simulink model "eml_hdl_design_patterns"  (R2026a)
settings: Solver=FixedStepDiscrete  StopTime=10
InitFcn:
  | errMsg  = ['\n\nThis model is only for demonstration purposes.\n\nPlease do not Simulate or code generate directly from this model. \n\nBefore generating code from this model please do copy the relevant blocks of interest from this model to a new model, place them in a subsystem, build a valid test bench around them.\n\nPlease refer to the example model ''eml_hdl_incrementer'' or HDLCoder documentation'];
  | error(sprintf(errMsg));
undefined symbols (not defined in the file or in its folder): C, gain_val, init_val, lower_limit, maxWordLength, thresh, upper_limit
libraries: simulink x2
(part 2 of 5)

== matlab function eml_hdl_design_patterns/Counters/counter_up_down_enable ==
  settings: fimath=|
      | fimath(...
      | 'RoundMode', 'floor',...
      | 'OverflowMode', 'wrap',...
      | 'ProductMode', 'FullPrecision', 'ProductWordLength', 32,...
      | 'SumMode', 'FullPrecision', 'SumWordLength', 32,...
      | 'CastBeforeSum', true)
  data: count output fixdt(0,4,0) size=1; up input boolean; down input boolean
function count = fcn(up, down)

% synchronous up down counter
% If "up" is set, it counts up.
% Else, if "down" is set, it counts down
% If neither is set it's disabled.

result_nt = numerictype(0,4,0);

% With "saturate" set this counter will never rollover.  To make it
% rollover, set the 'OverflowMode' to 'wrap'.
result_fm = fimath('OverflowMode', 'saturate', 'RoundMode', 'floor');

persistent count_reg;
if isempty(count_reg)
    count_reg = fi(0, result_nt, result_fm);
end

count = count_reg;

if up   
    inc = count_reg + fi(1, result_nt, result_fm);
    count_reg = fi(inc, result_nt, result_fm);
elseif down
    dec = count_reg - fi(1, result_nt, result_fm);
    count_reg = fi(dec, result_nt, result_fm);
end

== matlab function eml_hdl_design_patterns/Adders/full_adder ==
  settings: fimath=|
      | fimath(...
      | 'RoundMode', 'floor',...
      | 'OverflowMode', 'wrap',...
      | 'ProductMode', 'FullPrecision', 'ProductWordLength', 32,...
      | 'SumMode', 'FullPrecision', 'SumWordLength', 32,...
      | 'CastBeforeSum', true)
  data: a input fixdt(0,1,0); sum output; b input fixdt(0,1,0); cin input fixdt(0,1,0); cout output
function [sum,cout] = fcn(a, b, cin)

% Full Adder

% sum = (a^b)^cin
sum1 = bitxor(a,  b);
sum = bitxor(sum1, cin);

% cout = (a & b) | (b & cin) | (a & cin);
cout = bitor(bitor(bitand(a, b), bitand(b, cin)), bitand(a, cin));

== matlab function eml_hdl_design_patterns/Adders/unsigned_adder ==
  settings: fimath=|
      | fimath(...
      | 'RoundMode', 'floor',...
      | 'OverflowMode', 'wrap',...
      | 'ProductMode', 'FullPrecision', 'ProductWordLength', 32,...
      | 'SumMode', 'FullPrecision', 'SumWordLength', 32,...
      | 'CastBeforeSum', true)
  data: a input fixdt(0,3,0); sum output; b input fixdt(0,3,0)
function sum  = fcn(a, b)

% check default fimath settings on the block
% that define the following unsigned addition semantics
sum = a + b;

== matlab function eml_hdl_design_patterns/Adders/add_with_carry ==
  settings: fimath=|
      | fimath(...
      | 'RoundMode', 'floor',...
      | 'OverflowMode', 'wrap',...
      | 'ProductMode', 'FullPrecision', 'ProductWordLength', 32,...
      | 'SumMode', 'FullPrecision', 'SumWordLength', 32,...
      | 'CastBeforeSum', true)
  data: u1 input fixdt(1,5,0); sum output; u2 input fixdt(1,5,0); carry output; overflow output; c_in input fixdt(0,1,0); flags output
function [sum,carry,overflow,flags] = fcn(u1,u2,c_in)

% add with carry
% generates various CPU flags found in a FLAG register

nt_u1 = numerictype(u1);
fm_u1 = fimath(u1);

wlen  = nt_u1.WordLength;
ufix1_nt = numerictype(0, 1, 0);

% zero extend u1 by a bit
t_u1 = fi(u1, 1, wlen+1, 0);
t_u1 = bitset(t_u1, wlen+1, 0);

% zero extend u2 by a bit
t_u2 = fi(u2, 1, wlen+1, 0);
t_u2 = bitset(t_u2, wlen+1, 0);

% perform the addition
temp_sum = fi(t_u1+t_u2+c_in, 1, wlen+1, 0, fm_u1);

% Carry Flag (get msb)
carry = bitsliceget(temp_sum, wlen+1, wlen+1);

% Extract actual Sum
sum = fi(temp_sum, 1, wlen, 0, fm_u1);

% Negativity flag (N)
msb = getmsb(sum);

% Overflow Flag (V)
u1msb = getmsb(u1);
u2msb = getmsb(u2);
if((u1msb == u2msb) && (msb ~= u1msb))
    overflow = fi(1, ufix1_nt, fm_u1);
else
    overflow = fi(0, ufix1_nt, fm_u1);
end

if (all(sum))    
    zero = fi(1, 0, 1, 0);
else
    zero = fi(0, 0, 1, 0);
end

 
% construct the flag register
% flags = 'C N V Z'
flags = bitconcat(bitconcat(bitconcat(carry, msb), overflow), zero);

== matlab function eml_hdl_design_patterns/Adders/sub_with_borrow ==
  settings: fimath=|
      | fimath(...
      | 'RoundMode', 'floor',...
      | 'OverflowMode', 'wrap',...
      | 'ProductMode', 'FullPrecision', 'ProductWordLength', 32,...
      | 'SumMode', 'FullPrecision', 'SumWordLength', 32,...
      | 'CastBeforeSum', true)
  data: diff output; borrow output; u1 input fixdt(1,5,0); u2 input fixdt(1,5,0); overflow output; c_in input fixdt(0,1,0); flags output
function [diff,borrow,overflow,flags] = fcn(u1,u2,c_in)
% Implement add with carry using subtract with borrow

[diff,borrow,overflow,flags] = add_w_carry(u1,bitcmp(u2),bitcmp(c_in));


function [sum,carry,overflow,flags] = add_w_carry(u1,u2,c_in)

% add with carry
% generates various CPU flags found in a FLAG register

nt_u1 = numerictype(u1);
fm_u1 = fimath(u1);

wlen  = nt_u1.WordLength;
ufix1_nt = numerictype(0, 1, 0);

% zero extend u1 by a bit
t_u1 = fi(u1, 1, wlen+1, 0);
t_u1 = bitset(t_u1, wlen+1, 0);

% zero extend u2 by a bit
t_u2 = fi(u2, 1, wlen+1, 0);
t_u2 = bitset(t_u2, wlen+1, 0);

% perform the addition
temp_sum = fi(t_u1+t_u2+c_in, 1, wlen+1, 0, fm_u1);

% Carry Flag (get msb)
carry = bitsliceget(temp_sum, wlen+1, wlen+1);

% Extract actual Sum
sum = fi(temp_sum, 1, wlen, 0, fm_u1);

% Negativity flag (N)
msb = getmsb(sum);

% Overflow Flag (V)
u1msb = getmsb(u1);
u2msb = getmsb(u2);
if((u1msb == u2msb) && (msb ~= u1msb))
    overflow = fi(1, ufix1_nt, fm_u1);
else
    overflow = fi(0, ufix1_nt, fm_u1);
end

if (all(sum))    
    zero = fi(1, 0, 1, 0);
else
    zero = fi(0, 0, 1, 0);
end

 
% construct the flag register
% flags = 'C N V Z'
flags = bitconcat(bitconcat(bitconcat(carry, msb), overflow), zero);

== matlab function eml_hdl_design_patterns/Shift Registers/shift_reg_1by32 ==
  settings: fimath=|
      | fimath(...
      | 'RoundMode', 'floor',...
      | 'OverflowMode', 'wrap',...
      | 'ProductMode', 'FullPrecision', 'ProductWordLength', 32,...
      | 'SumMode', 'FullPrecision', 'SumWordLength', 32,...
      | 'CastBeforeSum', true)
  data: shift input boolean; sr_out output fixdt(0,1,0); sr_in input fixdt(0,1,0)
function sr_out = fcn(shift, sr_in)
%shift register 1 by 32

persistent sr;
if isempty(sr)
    sr = fi(0, 0, 32, 0, 'fimath', fimath(sr_in));
end

% return sr[31]
sr_out = getmsb(sr);

if (shift)
    % sr_new[32:1] = sr[31:1] & sr_in
    sr = bitconcat(bitsliceget(sr, 31, 1), sr_in);
end

== matlab function eml_hdl_design_patterns/FSMs/moore_fsm ==
  settings: fimath=|
      | fimath(...
      | 'RoundMode', 'nearest',...
      | 'OverflowMode', 'saturate',...
      | 'ProductMode', 'FullPrecision', 'ProductWordLength', 128,...
      | 'SumMode', 'FullPrecision', 'SumWordLength', 128,...
      | 'CastBeforeSum', true)
  data: A input boolean; Z output boolean size=1
function Z = fcn(A)

persistent moore_state_reg;
if isempty(moore_state_reg)
    moore_state_reg = fi(0, 0, 2, 0);   
end

S1 = 0;
S2 = 1;
S3 = 2;
S4 = 3;

switch (moore_state_reg)
    
    case S1
        
        Z = true;
        if (~A)
            moore_state_reg(1) = S1;
        else
            moore_state_reg(1) = S2;
        end
        
    case S2
        
        Z = false;
        if (~A)
            moore_state_reg(1) = S1;
        else
            moore_state_reg(1) = S2;
        end
        
    case S3
        
        Z = false;
        if (~A)
            moore_state_reg(1) = S2;
        else
            moore_state_reg(1) = S3;
        end
        
    case S4
        
        Z = true;
        if (~A)
            moore_state_reg(1) = S1;
        else
            moore_state_reg(1) = S3;
        end
    otherwise
        Z = false;
end

== matlab function eml_hdl_design_patterns/Shift Registers/shift_reg_1by64 ==
  settings: fimath=|
      | fimath(...
      | 'RoundMode', 'floor',...
      | 'OverflowMode', 'wrap',...
      | 'ProductMode', 'FullPrecision', 'ProductWordLength', 32,...
      | 'SumMode', 'FullPrecision', 'SumWordLength', 32,...
      | 'CastBeforeSum', true)
  data: shift input boolean; sr_tap1 output fixdt(0,1,0); sr_in input fixdt(0,1,0); sr_tap2 output
function [sr_tap1,sr_tap2] = fcn(shift, sr_in)

% mimimcing 64bit shift reg, using 32bit word due to
% our fixpt 32bit limitation.

persistent sr_lsw;
persistent sr_msw;

if isempty(sr_lsw)
    sr_lsw = fi(0, 0, 32, 0, 'fimath', fimath(sr_in));
    sr_msw = fi(0, 0, 32, 0, 'fimath', fimath(sr_in));    
end

% return sr_lsw[31]
sr_tap1 = getmsb(sr_lsw);
% return sr_msw[31]
sr_tap2 = getmsb(sr_msw);

if (shift)
    % sr_msw[31:1] = sr_msw[30:0] & sl_lsw[31]
    sr_msw = bitconcat(bitsliceget(sr_msw, 31, 1), getmsb(sr_lsw));
    % sr_lsw[31:1] = sr_lsw[30:0] & sr_in
    sr_lsw = bitconcat(bitsliceget(sr_lsw, 31, 1), sr_in);    
end

== matlab function eml_hdl_design_patterns/Signal Analysis/conv_output_side ==
  settings: fimath=|
      | fimath(...
      | 'RoundMode', 'floor',...
      | 'OverflowMode', 'wrap',...
      | 'ProductMode', 'FullPrecision', 'ProductWordLength', 32,...
      | 'SumMode', 'FullPrecision', 'SumWordLength', 32,...
      | 'CastBeforeSum', true)
  data: u input fixdt(0,6,2) size=80; y output; h input fixdt(0,6,2) size=30
function y = fcn(u, h)

% Convolution: on the output side

% this algorithm specifies how each sample in the output 
% signal can be calculated independently of all other samples 
% in the output signal.

% y has to be fully specified before indexing into it.
%  length(y) == 112, typeof(y) == ufix12_En6

nt = numerictype(0, 12, 6);
fm = fimath(u);

y = fi(zeros(1, 110), nt, fm);

for ii=1:110
    for jj=1:30
        kk = ii - jj;
        if kk >= 1 && kk <= 80
            y(kk) = fi(y(kk) + fi(h(jj) * u(kk), nt, fm), nt, fm);
        end
    end
end

== matlab function eml_hdl_design_patterns/Combinatorics/count_ones_blk ==
  settings: fimath=|
      | fimath(...
      | 'RoundMode', 'floor',...
      | 'OverflowMode', 'wrap',...
      | 'ProductMode', 'FullPrecision', 'ProductWordLength', 32,...
      | 'SumMode', 'FullPrecision', 'SumWordLength', 32,...
      | 'CastBeforeSum', true)
  data: datain input fixdt(0,17,0); result output fixdt(0,18,0) size=1
function result  = fcn(datain)

t = count_bits_in_range(datain);

r_nt = numerictype(0, 18, 0); 
r_fm = fimath('OverflowMode', 'saturate', 'RoundMode', 'floor');

result = fi(t, r_nt, r_fm);

%%%%%%%%%%%%%%%%%%%%%%%%%%%%%%%%%%%%%
% subfunction, counts bits in range
%%%%%%%%%%%%%%%%%%%%%%%%%%%%%%%%%%%%%
function cntOnes = count_bits_in_range(datain)

lbound = 1;
rbound = 17; % wlen of datain

cntOnes = uint8(0);

for ii=lbound:1:rbound
    bit = bitget(datain, ii);
    if logical(bit)
        cntOnes = cntOnes + 1;
    end
end

== matlab function eml_hdl_design_patterns/Misc/saturate_input ==
  data: u input; y output
function y = fcn(u) 
% Implementation of Saturation block with MATLAB code.

% Note Input can be integer or fixedpoint type 
% (see this block setting: treat input as int or fi)


upper_limit = fi(500, numerictype(u), fimath(u));
lower_limit = fi(-500, numerictype(u), fimath(u));

if (u > upper_limit)
    y = upper_limit;
elseif (u < lower_limit)
    y = lower_limit;
else
    y = u;
end

== matlab function eml_hdl_design_patterns/Word Twiddlers/nibble_swap_with_bitops ==
  settings: fimath=|
      | fimath(...
      | 'RoundMode', 'floor',...
      | 'OverflowMode', 'wrap',...
      | 'ProductMode', 'FullPrecision', 'ProductWordLength', 32,...
      | 'SumMode', 'FullPrecision', 'SumWordLength', 32,...
      | 'CastBeforeSum', true)
  data: u input fixdt(0,8,0); y output
function y = fcn(u)
% NIBBLE SWAP (using traditional bitops)

% assumes u is of type ufix8
% lmask = 0x0F
lmask = fi(15, 0, 8, 0, 'fimath', fimath(u));
% lmask = 0xF0
umask = bitsll(lmask, 4);
% mask upper nibble
l_nibble = bitand(u, lmask);
% mask lower nibble
u_nibble = bitand(u, umask);
% shift lower nibble left
ls = bitsll(l_nibble, 4);
% shift upper nibble right
ur = bitsrl(u_nibble, 4);
% final output
y = bitor(ls, ur);

== matlab function eml_hdl_design_patterns/Word Twiddlers/nibble_swap_with_slice_concat ==
  settings: fimath=|
      | fimath(...
      | 'RoundMode', 'floor',...
      | 'OverflowMode', 'wrap',...
      | 'ProductMode', 'FullPrecision', 'ProductWordLength', 32,...
      | 'SumMode', 'FullPrecision', 'SumWordLength', 32,...
      | 'CastBeforeSum', true)
  data: u input fixdt(0,8,0); y output
function y = fcn(u)
% NIBBLE SWAP
y = bitconcat(bitsliceget(u, 4, 1), bitsliceget(u, 8, 5));

== matlab function eml_hdl_design_patterns/Bit Twiddlers/hdl_bit_ops ==
  settings: fimath=|
      | fimath(...
      | 'RoundMode', 'floor',...
      | 'OverflowMode', 'saturate',...
      | 'ProductMode', 'FullPrecision', 'ProductWordLength', 32,...
      | 'SumMode', 'FullPrecision', 'SumWordLength', 32,...
      | 'CastBeforeSum', true)
  data: a input fixdt(0,31,0); b input fixdt(0,31,0); bget output; bslice output; bmsb output; blsb output; bset output; bcmp output; band output; bor output; bxor output; bnand output; bnor output; bnxor output; blshift output; brshift output; band_red output; bor_red output; bxor_red output; bnand_red output; bnor_red output; bnxor_red output
function [...
    bget, bslice, bmsb, blsb,...
    bset, bcmp,...
    band, bor, bxor, ...
    bnand, bnor, bnxor, ...
    blshift, brshift,  ...
    band_red, bor_red, bxor_red, ...
    bnand_red, bnor_red, bnxor_red] = fcn(a,b)


% BITGET
% get bit at position of fixed point input var 'a'
% this uses slice operator in HDL
bget = bitget(a,2);
bslice = bitsliceget(a, 25, 20);
bmsb = getmsb(a);
blsb = getlsb(a);

% BITCLEAR
% clear bit at position 3 and compute new value into 't2'
t2 = bitset(a,3,0);

% BITSET
% now set bit4 in t2
% you need to assign the result back to 't2' to update the variable
bset = bitset(t2,4,1);

% BITCMP
bcmp = bitcmp(a);

% BITAND
band = bitand(a,b);
% BITOR
bor = bitor(a,b);
% BITXOR
bxor = bitxor(a,b);

% BITNAND
bnand = bitcmp(bitand(a,b));
% BITNOR
bnor = bitcmp(bitor(a,b));
% NOT BITXOR
bnxor = bitcmp(bitxor(a,b));

% BITSHIFT
% multitply by 2
blshift = bitsll(a,1); 
% divide by 2
brshift = bitsrl(a,1); 

% AND, XOR, OR REDUCTION 
band_red = bitandreduce(a);
bxor_red = bitxorreduce(a);
bor_red = bitorreduce(a);

% NAND, NOR, NOT XOR, REDUCTION 
bnand_red = bitcmp(band_red);
bnxor_red = bitcmp(bxor_red);
bnor_red = bitcmp(bor_red);

== matlab function eml_hdl_design_patterns/Shift Registers/shift_reg_universal ==
  settings: fimath=|
      | fimath(...
      | 'RoundMode', 'nearest',...
      | 'OverflowMode', 'saturate',...
      | 'ProductMode', 'FullPrecision', 'ProductWordLength', 128,...
      | 'SumMode', 'FullPrecision', 'SumWordLength', 128,...
      | 'CastBeforeSum', true)
  data: Clear input boolean; Q output fixdt(0,3,0) size=1; LeftIn input boolean; RightIn input boolean; S1 input boolean; S2 input boolean; InData input fixdt(0,3,0)
function Q = fcn(Clear, LeftIn, RightIn, S1, S2, InData)

% 3bit universal shift register. it can
%  a) hold value
%  b) shift left
%  c) shift right
%  d) load value

% this can be used as
%  serial-in, serial-out shift reg
%  parallel-in, serial-out shift reg
%  serial-in, parallel-out shift reg
%  parallel-in, parallel-out shift reg

% state table

% --------------------------------------------------------
% function        inputs          next state
%                 S1, S2          Q2 Q1 Q0
% --------------------------------------------------------
% hold            0   0           Q2      Q1      Q0
% shift left      0   1           Q1      Q0      RightIn
% shift right     1   0           LeftIn  Q2      Q1
% load            1   1           in2     in1     in0
% --------------------------------------------------------

persistent Q_reg;
if isempty(Q_reg)
    Q_reg = fi(0, 0, 3, 0);
end

Q = Q_reg;
if Clear
    Q = fi(0, 0, 3, 0);
else
    switch uint8(S1)

        case 0
            switch uint8(S2)
                case 0
                    % state: 00
                    % do nothing
                case 1
                    % state: 01
                    % shift left, and feed datain from right
                    Q_reg = bitsll(Q_reg, 1);
                    Q_reg = bitset(Q_reg, 1, RightIn);
            end

        case 1
            switch uint8(S2)
                case 0
                    % state: 10
                    % shift right, and feed datain from left
                    Q_reg = bitsrl(Q_reg, 1);
                    Q_reg = bitset(Q_reg, 3, LeftIn);
                case 1
                    % state: 11
                    % load value
                    Q_reg = InData;
            end
    end
end

== matlab function eml_hdl_design_patterns/Decoders/monlithic_viterbi ==
  settings: fimath=|
      | fimath(...
      | 'RoundMode', 'floor',...
      | 'OverflowMode', 'wrap',...
      | 'ProductMode', 'FullPrecision', 'ProductWordLength', 32,...
      | 'SumMode', 'FullPrecision', 'SumWordLength', 32,...
      | 'CastBeforeSum', true)
  data: u input fixdt(1,6,3) size=2; y output boolean
function y = fcn(u)
%--------------------------------------------------------------------------
% Viterbi Decoder Demo
% 
% This model implements viterbi decoder with a MATLAB Function Block.
% The Viterbi Decoder block decodes fixed-point input symbols to produce 
% binary output symbols.
%--------------------------------------------------------------------------

% stored paths metrics register
persistent sm_reg;  
if isempty(sm_reg)
    sm_reg = getfi_sat(zeros(1,64),1, 12, 6);
end

% traceback storage register
persistent tb_reg;  
if isempty(tb_reg)
    tb_reg = getfi(zeros(1,64), 0, 27, 0);
end

% traceback output register
persistent tbout_reg
if isempty(tbout_reg)
    tbout_reg = getfi(0,0,1,0);
end

% input symbol
u1 = u(1);
u2 = u(2);

%--------------------------------------------------------------------------
% BMC (Branch Metric) Unit
% This block calculates the Branch Metric (Hamming distance) of input symbols.
% The input are the quantized fixed-point symbols in the form of sfix6_En3.
%--------------------------------------------------------------------------
bm = getfi_sat(zeros(1,4), 1, 12, 6);

%----------------------------
% Hamming distace for (1,1)
%----------------------------
bm(1) = (u1-1)*(u1-1) + (u2-1)*(u2-1);

%----------------------------
% Hamming distace for (1,-1)
%----------------------------
bm(2) = (u1-1)*(u1-1) + (u2-(-1))*(u2-(-1));

%----------------------------
% Hamming distace for (-1,1)
%----------------------------
bm(3) = (u1-(-1))*(u1-(-1)) + (u2-1)*(u2-1);

%----------------------------
% Hamming distace for (-1,-1)
%----------------------------
bm(4) = (u1-(-1))*(u1-(-1)) + (u2-(-1))*(u2-(-1));

%--------------------------------------------------------------------------
% PMU (Path Metric Unit)
% This block calculates and compares the path metrics to get the optimal path.
% The core elements of this block are 
%  a) ACS (Add-Compare-Select) block, and 
%  b) Renormalize block
%--------------------------------------------------------------------------

% ACS Unit Group Block
[nsm, dec] = acsunitbutterfly(bm, sm_reg);

% Renormalize Block
% Finds the state with minimum path metric and outputs its index
% Then renormalizes all the path metrics by subsracting the minimum metric
[minimum, idx] = tree_min(nsm);
index = getfi((idx-1), 0, 8, 0);
sm_reg = getfi_sat((nsm - minimum), 1, 12, 6);
    
%--------------------------------------------------------------------------
% TBU (Trace Back Unit)
% Trace back unit restore the optimal path information stored in the 
% path metric register. The trace back depth of this decoder is 32 steps,
% which means every decoded symbol is based on the minimum path metric in the
% following 32 steps. 
%
% The trace back unit is implemented by a 27 stage shift register.
% Only 27 stage is necessary (instead of 32) because we can retrieve the 
% input symbol of the 32th stage from the shift register index of the 27th stage.
%
% Normal implementation uses 27 64-bit registers for trance back unit. 
% We use 64 27-bit registers instead because of the fixed-point bitwidth limit.
%--------------------------------------------------------------------------

% stores path metric decision inforamtion from PMU unit
tb_reg = bitshift(tb_reg, 1);
tb_reg = bitset(tb_reg, ones(1,64), uint8(dec));

% trace back unit
for i=1:27
  index = tbunit(index, tb_reg, i);
end

% the LSB of the 27th trace back step is the decoder output
tbmask = getfi(1, 0, 8, 0);
tband = bitand(index, tbmask);

% register the final result
prev_result = tbout_reg;
tbout_reg = getfi(tband, 0, 1, 0);

% update output as boolean datatype
y =  (prev_result == getfi(1, 0, 1, 0));

end

%--------------------------------------------------------------------------
% TB Unit (Trace Back Unit)
% Given the index of the minimum metric node in the current stages,
% also given the stored decision information in the current stages,
% we can restore the index of the minimum metric node in the previous stage.
%--------------------------------------------------------------------------
function new_idx = tbunit (current_idx, tb_reg, stage)

idx = int8(current_idx) + int8(1);
tbread = bitget(tb_reg(idx), stage);

tbshift = bitshift(current_idx, 1);
tband = bitand(tbshift, getfi(62, 0, 8, 0));
new_idx = bitor(tband, getfi(tbread, 0, 8, 0));

end

%--------------------------------------------------------------------------
% ACS Unit Group(Add-Compare-Select)
% For each state in the trellis diagram, for each node in this state:
% 1. Add the branch metric to the paths merged to this node. 
% 2. Compare all the paths merged to this road
% 3. Select the path with the minimum path metric
%
% The following code is generated by a script 'generateviterbi.m'
% that generates trellis diagram for convolution code (7,171,133)
%--------------------------------------------------------------------------
function [nsm, dec] = acsunitbutterfly(bm, sm)

nsm = getfi(zeros(1,64),1, 12, 6);
dec = getfi(zeros(1,64),0, 1,  0);

%----------------------------------------------------
% 000000   -> 00 -> 000000   000001   -> 11 -> 000000   
%----------------------------------------------------
[nsm(1), dec(1)] = acsunit(bm(1),bm(4),sm(1),sm(2));
%----------------------------------------------------
% 000000   -> 11 -> 100000   000001   -> 00 -> 100000   
%----------------------------------------------------
[nsm(33), dec(33)] = acsunit(bm(4),bm(1),sm(1),sm(2));
%----------------------------------------------------
% 000010   -> 01 -> 000001   000011   -> 10 -> 000001   
%----------------------------------------------------
[nsm(2), dec(2)] = acsunit(bm(2),bm(3),sm(3),sm(4));
%----------------------------------------------------
% 000010   -> 10 -> 100001   000011   -> 01 -> 100001   
%----------------------------------------------------
[nsm(34), dec(34)] = acsunit(bm(3),bm(2),sm(3),sm(4));
%----------------------------------------------------
% 000100   -> 00 -> 000010   000101   -> 11 -> 000010   
%----------------------------------------------------
[nsm(3), dec(3)] = acsunit(bm(1),bm(4),sm(5),sm(6));
%----------------------------------------------------
% 000100   -> 11 -> 100010   000101   -> 00 -> 100010   
%----------------------------------------------------
[nsm(35), dec(35)] = acsunit(bm(4),bm(1),sm(5),sm(6));
%----------------------------------------------------
% 000110   -> 01 -> 000011   000111   -> 10 -> 000011   
%----------------------------------------------------
[nsm(4), dec(4)] = acsunit(bm(2),bm(3),sm(7),sm(8));
%----------------------------------------------------
% 000110   -> 10 -> 100011   000111   -> 01 -> 100011   
%----------------------------------------------------
[nsm(36), dec(36)] = acsunit(bm(3),bm(2),sm(7),sm(8));
%----------------------------------------------------
% 001000   -> 11 -> 000100   001001   -> 00 -> 000100   
%----------------------------------------------------
[nsm(5), dec(5)] = acsunit(bm(4),bm(1),sm(9),sm(10));
%----------------------------------------------------
% 001000   -> 00 -> 100100   001001   -> 11 -> 100100   
%----------------------------------------------------
[nsm(37), dec(37)] = acsunit(bm(1),bm(4),sm(9),sm(10));
%----------------------------------------------------
% 001010   -> 10 -> 000101   001011   -> 01 -> 000101   
%----------------------------------------------------
[nsm(6), dec(6)] = acsunit(bm(3),bm(2),sm(11),sm(12));
%----------------------------------------------------
% 001010   -> 01 -> 100101   001011   -> 10 -> 100101   
%----------------------------------------------------
[nsm(38), dec(38)] = acsunit(bm(2),bm(3),sm(11),sm(12));
%----------------------------------------------------
% 001100   -> 11 -> 000110   001101   -> 00 -> 000110   
%----------------------------------------------------
[nsm(7), dec(7)] = acsunit(bm(4),bm(1),sm(13),sm(14));
%----------------------------------------------------
% 001100   -> 00 -> 100110   001101   -> 11 -> 100110   
%----------------------------------------------------
[nsm(39), dec(39)] = acsunit(bm(1),bm(4),sm(13),sm(14));
%----------------------------------------------------
% 001110   -> 10 -> 000111   001111   -> 01 -> 000111   
%----------------------------------------------------
[nsm(8), dec(8)] = acsunit(bm(3),bm(2),sm(15),sm(16));
%----------------------------------------------------
% 001110   -> 01 -> 100111   001111   -> 10 -> 100111   
%----------------------------------------------------
[nsm(40), dec(40)] = acsunit(bm(2),bm(3),sm(15),sm(16));
%----------------------------------------------------
% 010000   -> 11 -> 001000   010001   -> 00 -> 001000   
%----------------------------------------------------
[nsm(9), dec(9)] = acsunit(bm(4),bm(1),sm(17),sm(18));
%----------------------------------------------------
% 010000   -> 00 -> 101000   010001   -> 11 -> 101000   
%----------------------------------------------------
[nsm(41), dec(41)] = acsunit(bm(1),bm(4),sm(17),sm(18));
%----------------------------------------------------
% 010010   -> 10 -> 001001   010011   -> 01 -> 001001   
%----------------------------------------------------
[nsm(10), dec(10)] = acsunit(bm(3),bm(2),sm(19),sm(20));
%----------------------------------------------------
% 010010   -> 01 -> 101001   010011   -> 10 -> 101001   
%----------------------------------------------------
[nsm(42), dec(42)] = acsunit(bm(2),bm(3),sm(19),sm(20));
%----------------------------------------------------
% 010100   -> 11 -> 001010   010101   -> 00 -> 001010   
%----------------------------------------------------
[nsm(11), dec(11)] = acsunit(bm(4),bm(1),sm(21),sm(22));
%----------------------------------------------------
% 010100   -> 00 -> 101010   010101   -> 11 -> 101010   
%----------------------------------------------------
[nsm(43), dec(43)] = acsunit(bm(1),bm(4),sm(21),sm(22));
%----------------------------------------------------
% 010110   -> 10 -> 001011   010111   -> 01 -> 001011   
%----------------------------------------------------
[nsm(12), dec(12)] = acsunit(bm(3),bm(2),sm(23),sm(24));
%----------------------------------------------------
% 010110   -> 01 -> 101011   010111   -> 10 -> 101011   
%----------------------------------------------------
[nsm(44), dec(44)] = acsunit(bm(2),bm(3),sm(23),sm(24));
%----------------------------------------------------
% 011000   -> 00 -> 001100   011001   -> 11 -> 001100   
%----------------------------------------------------
[nsm(13), dec(13)] = acsunit(bm(1),bm(4),sm(25),sm(26));
%----------------------------------------------------
% 011000   -> 11 -> 101100   011001   -> 00 -> 101100   
%----------------------------------------------------
[nsm(45), dec(45)] = acsunit(bm(4),bm(1),sm(25),sm(26));
%----------------------------------------------------
% 011010   -> 01 -> 001101   011011   -> 10 -> 001101   
%----------------------------------------------------
[nsm(14), dec(14)] = acsunit(bm(2),bm(3),sm(27),sm(28));
%----------------------------------------------------
% 011010   -> 10 -> 101101   011011   -> 01 -> 101101   
%----------------------------------------------------
[nsm(46), dec(46)] = acsunit(bm(3),bm(2),sm(27),sm(28));
%----------------------------------------------------
% 011100   -> 00 -> 001110   011101   -> 11 -> 001110   
%----------------------------------------------------
[nsm(15), dec(15)] = acsunit(bm(1),bm(4),sm(29),sm(30));
%----------------------------------------------------
% 011100   -> 11 -> 101110   011101   -> 00 -> 101110   
%----------------------------------------------------
[nsm(47), dec(47)] = acsunit(bm(4),bm(1),sm(29),sm(30));
%----------------------------------------------------
% 011110   -> 01 -> 001111   011111   -> 10 -> 001111   
%----------------------------------------------------
[nsm(16), dec(16)] = acsunit(bm(2),bm(3),sm(31),sm(32));
%----------------------------------------------------
% 011110   -> 10 -> 101111   011111   -> 01 -> 101111   
%----------------------------------------------------
[nsm(48), dec(48)] = acsunit(bm(3),bm(2),sm(31),sm(32));
%----------------------------------------------------
% 100000   -> 10 -> 010000   100001   -> 01 -> 010000   
%----------------------------------------------------
[nsm(17), dec(17)] = acsunit(bm(3),bm(2),sm(33),sm(34));
%----------------------------------------------------
% 100000   -> 01 -> 110000   100001   -> 10 -> 110000   
%----------------------------------------------------
[nsm(49), dec(49)] = acsunit(bm(2),bm(3),sm(33),sm(34));
%----------------------------------------------------
% 100010   -> 11 -> 010001   100011   -> 00 -> 010001   
%----------------------------------------------------
[nsm(18), dec(18)] = acsunit(bm(4),bm(1),sm(35),sm(36));
%----------------------------------------------------
% 100010   -> 00 -> 110001   100011   -> 11 -> 110001   
%----------------------------------------------------
[nsm(50), dec(50)] = acsunit(bm(1),bm(4),sm(35),sm(36));
%----------------------------------------------------
% 100100   -> 10 -> 010010   100101   -> 01 -> 010010   
%----------------------------------------------------
[nsm(19), dec(19)] = acsunit(bm(3),bm(2),sm(37),sm(38));
%----------------------------------------------------
% 100100   -> 01 -> 110010   100101   -> 10 -> 110010   
%----------------------------------------------------
[nsm(51), dec(51)] = acsunit(bm(2),bm(3),sm(37),sm(38));
%----------------------------------------------------
% 100110   -> 11 -> 010011   100111   -> 00 -> 010011   
%----------------------------------------------------
[nsm(20), dec(20)] = acsunit(bm(4),bm(1),sm(39),sm(40));
%----------------------------------------------------
% 100110   -> 00 -> 110011   100111   -> 11 -> 110011   
%----------------------------------------------------
[nsm(52), dec(52)] = acsunit(bm(1),bm(4),sm(39),sm(40));
%----------------------------------------------------
% 101000   -> 01 -> 010100   101001   -> 10 -> 010100   
%----------------------------------------------------
[nsm(21), dec(21)] = acsunit(bm(2),bm(3),sm(41),sm(42));
%----------------------------------------------------
% 101000   -> 10 -> 110100   101001   -> 01 -> 110100   
%----------------------------------------------------
[nsm(53), dec(53)] = acsunit(bm(3),bm(2),sm(41),sm(42));
%----------------------------------------------------
% 101010   -> 00 -> 010101   101011   -> 11 -> 010101   
%----------------------------------------------------
[nsm(22), dec(22)] = acsunit(bm(1),bm(4),sm(43),sm(44));
%----------------------------------------------------
% 101010   -> 11 -> 110101   101011   -> 00 -> 110101   
%----------------------------------------------------
[nsm(54), dec(54)] = acsunit(bm(4),bm(1),sm(43),sm(44));
%----------------------------------------------------
% 101100   -> 01 -> 010110   101101   -> 10 -> 010110   
%----------------------------------------------------
[nsm(23), dec(23)] = acsunit(bm(2),bm(3),sm(45),sm(46));
%----------------------------------------------------
% 101100   -> 10 -> 110110   101101   -> 01 -> 110110   
%----------------------------------------------------
[nsm(55), dec(55)] = acsunit(bm(3),bm(2),sm(45),sm(46));
%----------------------------------------------------
% 101110   -> 00 -> 010111   101111   -> 11 -> 010111   
%----------------------------------------------------
[nsm(24), dec(24)] = acsunit(bm(1),bm(4),sm(47),sm(48));
%----------------------------------------------------
% 101110   -> 11 -> 110111   101111   -> 00 -> 110111   
%----------------------------------------------------
[nsm(56), dec(56)] = acsunit(bm(4),bm(1),sm(47),sm(48));
%----------------------------------------------------
% 110000   -> 01 -> 011000   110001   -> 10 -> 011000   
%----------------------------------------------------
[nsm(25), dec(25)] = acsunit(bm(2),bm(3),sm(49),sm(50));
%----------------------------------------------------
% 110000   -> 10 -> 111000   110001   -> 01 -> 111000   
%----------------------------------------------------
[nsm(57), dec(57)] = acsunit(bm(3),bm(2),sm(49),sm(50));
%----------------------------------------------------
% 110010   -> 00 -> 011001   110011   -> 11 -> 011001   
%----------------------------------------------------
[nsm(26), dec(26)] = acsunit(bm(1),bm(4),sm(51),sm(52));
%----------------------------------------------------
% 110010   -> 11 -> 111001   110011   -> 00 -> 111001   
%----------------------------------------------------
[nsm(58), dec(58)] = acsunit(bm(4),bm(1),sm(51),sm(52));
%----------------------------------------------------
% 110100   -> 01 -> 011010   110101   -> 10 -> 011010   
%----------------------------------------------------
[nsm(27), dec(27)] = acsunit(bm(2),bm(3),sm(53),sm(54));
%----------------------------------------------------
% 110100   -> 10 -> 111010   110101   -> 01 -> 111010   
%----------------------------------------------------
[nsm(59), dec(59)] = acsunit(bm(3),bm(2),sm(53),sm(54));
%----------------------------------------------------
% 110110   -> 00 -> 011011   110111   -> 11 -> 011011   
%----------------------------------------------------
[nsm(28), dec(28)] = acsunit(bm(1),bm(4),sm(55),sm(56));
%----------------------------------------------------
% 110110   -> 11 -> 111011   110111   -> 00 -> 111011   
%----------------------------------------------------
[nsm(60), dec(60)] = acsunit(bm(4),bm(1),sm(55),sm(56));
%----------------------------------------------------
% 111000   -> 10 -> 011100   111001   -> 01 -> 011100   
%----------------------------------------------------
[nsm(29), dec(29)] = acsunit(bm(3),bm(2),sm(57),sm(58));
%----------------------------------------------------
% 111000   -> 01 -> 111100   111001   -> 10 -> 111100   
%----------------------------------------------------
[nsm(61), dec(61)] = acsunit(bm(2),bm(3),sm(57),sm(58));
%----------------------------------------------------
% 111010   -> 11 -> 011101   111011   -> 00 -> 011101   
%----------------------------------------------------
[nsm(30), dec(30)] = acsunit(bm(4),bm(1),sm(59),sm(60));
%----------------------------------------------------
% 111010   -> 00 -> 111101   111011   -> 11 -> 111101   
%----------------------------------------------------
[nsm(62), dec(62)] = acsunit(bm(1),bm(4),sm(59),sm(60));
%----------------------------------------------------
% 111100   -> 10 -> 011110   111101   -> 01 -> 011110   
%----------------------------------------------------
[nsm(31), dec(31)] = acsunit(bm(3),bm(2),sm(61),sm(62));
%----------------------------------------------------
% 111100   -> 01 -> 111110   111101   -> 10 -> 111110   
%----------------------------------------------------
[nsm(63), dec(63)] = acsunit(bm(2),bm(3),sm(61),sm(62));
%----------------------------------------------------
% 111110   -> 11 -> 011111   111111   -> 00 -> 011111   
%----------------------------------------------------
[nsm(32), dec(32)] = acsunit(bm(4),bm(1),sm(63),sm(64));
%----------------------------------------------------
% 111110   -> 00 -> 111111   111111   -> 11 -> 111111   
%----------------------------------------------------
[nsm(64), dec(64)] = acsunit(bm(1),bm(4),sm(63),sm(64));

end    
    
% ACS unit
function [select_metric, decision] = acsunit(branch_metric0, branch_metric1, stored_metric0, stored_metric1)

    % update branch0 metric
    a = getfi_sat(branch_metric0 + stored_metric0, 1, 12, 6);

    % update branch1 metric
    b = getfi_sat(branch_metric1 + stored_metric1, 1, 12, 6);
    
    % choose the metric
    if (a <= b)
        select_metric = a;
        decision = getfi(0, 0, 1, 0);
    else
        select_metric = b;
        decision = getfi(1, 0, 1, 0);
    end
end
            
%--------------------------------------------------------------------------
% Tree implementation min function for vector input of length 64
%--------------------------------------------------------------------------
function [minval, idx] = tree_min(invec)

% initialize outputs
minval = getfi(0, 1, 12, 6);
idx = 0;

% first level of comparison
inidx = 1:64;
[lvlonemin, lvloneidx] = vector_min(invec, inidx);

% second level of comparison
[lvltwomin, lvltwoidx] = vector_min(lvlonemin, lvloneidx);

% third level of comparison
[lvlthreemin, lvlthreeidx] = vector_min(lvltwomin, lvltwoidx);

% fourth level of comparison
[lvlfourmin, lvlfouridx] = vector_min(lvlthreemin, lvlthreeidx);

% fifth level of comparison
[lvlfivemin, lvlfiveidx] = vector_min(lvlfourmin, lvlfouridx);

% final comparison
[minval, idx] = vector_min(lvlfivemin, lvlfiveidx);

end

% Minimum subfuction for tree implementation
function [minvec, idxvec] = vector_min(invec, inidx)
    
lengthminvec = uint8(length(invec)/2);
minvec = getfi(zeros(lengthminvec, 1), 1, 12, 6);
idxvec = zeros(lengthminvec, 1);

for i=1:lengthminvec
    % get two consecutive values
    idx2 = int8(i)+int8(i); %i*2
    idx1 = int8(idx2) - int8(1); %i*2-1
    % get elements
    val1 = invec(idx1);
    val2 = invec(idx2);
    % compare them and select minimum
    if le(val1, val2)
        minvec(i) = val1;
        idxvec(i) = inidx(idx1);
    else
        minvec(i) = val2;
        idxvec(i) = inidx(idx2);
    end
end

end


function myfi = getfi(input, issigned, wlen, flen)

fm = fimath(...
    'RoundMode', 'floor',...
    'OverflowMode', 'wrap',...
    'ProductMode', 'FullPrecision', 'ProductWordLength', 32,...
    'SumMode', 'FullPrecision', 'SumWordLength', 32,...
    'CastBeforeSum', true);

myfi = fi(input, issigned, wlen, flen, 'fimath', fm);

end


function myfi = getfi_sat(input, issigned, wlen, flen)

fm_sat = fimath(...
    'RoundMode', 'floor',...
    'OverflowMode', 'saturate',...
    'ProductMode', 'FullPrecision', 'ProductWordLength', 32,...
    'SumMode', 'FullPrecision', 'SumWordLength', 32,...
    'CastBeforeSum', true);

myfi = fi(input, issigned, wlen, flen, 'fimath', fm_sat);

end

== matlab function eml_hdl_design_patterns/Mux Demux/demux_using_for_blk ==
  settings: fimath=|
      | fimath(...
      | 'RoundMode', 'floor',...
      | 'OverflowMode', 'wrap',...
      | 'ProductMode', 'FullPrecision', 'ProductWordLength', 32,...
      | 'SumMode', 'FullPrecision', 'SumWordLength', 32,...
      | 'CastBeforeSum', true)
  data: address input uint8; line output fixdt(0,1,0) size=4
function line  = fcn(address)

line = fi(zeros(4, 1), 0, 1, 0);

for J=4:-1:1
    if (address == J)
        line(J) = 1;
    else
        line(J) = 0;
    end
end

== matlab function eml_hdl_design_patterns/Decoders/decoder_n_bit ==
  settings: fimath=|
      | fimath(...
      | 'RoundMode', 'floor',...
      | 'OverflowMode', 'wrap',...
      | 'ProductMode', 'FullPrecision', 'ProductWordLength', 32,...
      | 'SumMode', 'FullPrecision', 'SumWordLength', 32,...
      | 'CastBeforeSum', true)
  data: select_addr input boolean; decode_out output fixdt(0,1,0) size=4
function decode_out  = fcn(select_addr)

% N bit binary decoder

decode_out = fi(zeros(4,1), 0, 1, 0);

for jj = 4 : -1 : 1
    if jj == select_addr
        decode_out(jj) = fi(0, 0, 1, 0);
    else
        decode_out(jj) = fi(1, 0, 1, 0);
    end
end

== matlab function eml_hdl_design_patterns/Decoders/decoder_2_by_4 ==
  settings: fimath=|
      | fimath(...
      | 'RoundMode', 'floor',...
      | 'OverflowMode', 'wrap',...
      | 'ProductMode', 'FullPrecision', 'ProductWordLength', 32,...
      | 'SumMode', 'FullPrecision', 'SumWordLength', 32,...
      | 'CastBeforeSum', true)
  data: a input boolean; decode_out output fixdt(0,4,0) size=1; b input boolean; enable input boolean
function decode_out  = fcn(a, b, enable)

% 2 by 4 decoder circuit.

result_nt = numerictype(0,4,0);
result_fm = fimath('OverflowMode', 'wrap', 'RoundMode', 'floor');
decode_out = fi(0, result_nt, result_fm);

a_bar = ~a;
b_bar = ~b;

% compute bit0
decode_out = bitset(decode_out, 1, ~(enable & a_bar & b_bar));
% compute bit1
decode_out = bitset(decode_out, 2, ~(enable & a_bar & b));
% compute bit2
decode_out = bitset(decode_out, 3, ~(enable & a & b_bar));
% compute bit3
decode_out = bitset(decode_out, 4, ~(enable & a & b));

== matlab function eml_hdl_design_patterns/Combinatorics/pow2Test ==
  settings: fimath=|
      | fimath(...
      | 'RoundMode', 'floor',...
      | 'OverflowMode', 'wrap',...
      | 'ProductMode', 'FullPrecision', 'ProductWordLength', 32,...
      | 'SumMode', 'FullPrecision', 'SumWordLength', 32,...
      | 'CastBeforeSum', true)
  data: u input fixdt(0,6,0); y output
function y = fcn(u)
% y = ((u&(u-1))==0) ;
% (NB: This code sets 'b' to TRUE if 'n' is an integer power of two 
%  - in this context, both zero and one are considered to be powers of two.)
% 
% This code actually works by changing the 
% least significant '1' bit of 'n' to a '0'. If 'n' is a power of two, 
% it only has one '1' bit - and zeroing it leaves you with zero 
% as the answer.
% 
% Hence, the inner expression is also a cute trick... 


% couple of tweaks in this model to get good HDL out
% 1) change fimath on the block to use FullPrecision for Addition.
% 2) cast the result of subtraction (n-1) back to input type
%    (full precision subtraction results in a type which is one bit 
%     higher than sum of input word lengths. this is needed as 'bitand'
%     requires both inputs to be of same type.


inNT = numerictype(u);
inFM = fimath(u);

persistent allPowersOf2;
persistent index;
if isempty(allPowersOf2)
    index = 0;
    allPowersOf2 = fi(zeros(1, 32), inNT, inFM);
end

one = fi(1, inNT, inFM);
zero = fi(0, inNT, inFM);

u1 = u;
u2 = fi(u-one, inNT, inFM);

isPow2 = bitand(u1,u2) == zero;

if isPow2 && index<32
    allPowersOf2(index+1) = u;
    index = index+1;
end

y = allPowersOf2;

== matlab function eml_hdl_design_patterns/Filters/symmetric_fir ==
  settings: fimath=|
      | fimath(...
      | 'RoundMode', 'floor',...
      | 'OverflowMode', 'wrap',...
      | 'ProductMode', 'FullPrecision',...
      | 'SumMode', 'FullPrecision',...
      | 'CastBeforeSum', true)
  data: x_in input fixdt(1,6,0); y_out output; h_in1 input fixdt(1,6,0); h_in2 input fixdt(1,6,0); h_in3 input fixdt(1,6,0); h_in4 input fixdt(1,6,0)
function y_out  = fcn(x_in, h_in1, h_in2, h_in3, h_in4)
% This block supports an embeddable subset of the MATLAB language.
% See the help menu for details. 

persistent delay;

if isempty(delay)
    delay = fi(zeros(1,8), numerictype(x_in), fimath(x_in));
end

% add  delayed samples

%add val1 and val8
add1 = delay(1) + delay(8);

%add val2 and val7
add2 = delay(2) + delay(7);

%add val3 and val6
add3 = delay(3) + delay(6);

%add val4 and val5
add4 = delay(4) + delay(5);

% compute products
prod1 = add1 * h_in1;
prod2 = add2 * h_in2;
prod3 = add3 * h_in3;
prod4 = add4 * h_in4;

% compute final sums
add5 = prod1 + prod2;
add6 = prod3 + prod4;
add7 = add5 + add6;

y_out = add7;

% update pipeline
delay = [x_in delay(1:7)];

== matlab function eml_hdl_design_patterns/Word Twiddlers/Byte_ to_M_tuple ==
  data: u input uint8 size=204; y output fixdt(0,6,0)
function y = fcn(u)
% convert Bytes to M tuples

% This particular example uses bitwise slice and concat operations 
% to convert a frame of words 204x8 (bytes) to 272x6 (6bit tuples).

% The following algorithm works on 3 bytes at a time 

symbolWL    = 6; % Number of bits per M-ary symbol (word length), M = 64
inpFrameLen = length(u);
outFrameLen = 8*inpFrameLen / symbolWL;

% Initialize output index counter, dimensions, and data type
% ----------------------------------------------------------
out_idx = int32(1);
y       = fi(zeros(outFrameLen,1),0,6,0);

% Do the byte to m-tuple conversion
% ---------------------------------
nt = numerictype(0, 8, 0); % FI equivalent to uint8 (for bitwise ops below)
for inp_idx = int32(1:3:inpFrameLen)
    % Get next three (uint8) input words
    a = fi(u(inp_idx),   nt);
    b = fi(u(inp_idx+1), nt);
    c = fi(u(inp_idx+2), nt);
    
    % Form next four (ufix6) output words
    % starting with the MSB of the first word
    y(out_idx)   = bitsliceget(a, 8, 3);
    y(out_idx+1) = bitconcat(bitsliceget(a, 2, 1), bitsliceget(b, 8, 5));
    y(out_idx+2) = bitconcat(bitsliceget(b, 4, 1), bitsliceget(c, 8, 7));
    y(out_idx+3) = bitsliceget(c, 6, 1);
    
    % Increment out_idx for next time through loop
    out_idx = out_idx + 4;
end

== matlab function eml_hdl_design_patterns/Word Twiddlers/M_Tuple_ to_Byte ==
  data: u input fixdt(0,6,0) size=272; y output uint8
function y = fcn(u)
% convert M tuples to Bytes

% This particular example uses bitwise slice and concat operations 
% to convert a frame of words 272x6 (6bit tuples) to 204x8 (bytes).

% The following algorithm works on 4 tuples at a time 

inpFrameLen = length(u);
symbolWL    = 6; % Number of bits per M-ary symbol (word length), M = 64
outFrameLen = symbolWL*inpFrameLen / 8;

% Initialize output index counter, dimensions, and data type
% ----------------------------------------------------------
out_idx = int32(1);
% Use the FI equivalent to uint8 (for bitwise ops below)
yt = fi(zeros(outFrameLen,1), 0, 8, 0);

% Do the byte to m-tuple conversion
% ---------------------------------
for inp_idx = int32(1:4:inpFrameLen)
    % Get next four (ufix6) input words
    i1 = u(inp_idx);
    i2 = u(inp_idx+1);
    i3 = u(inp_idx+2);
    i4 = u(inp_idx+3);
    
    % Form next three (uint8) output words
    % starting with the MSB of the first word
    yt(out_idx)   = bitconcat(i1,                    bitsliceget(i2, 6, 5));
    yt(out_idx+1) = bitconcat(bitsliceget(i2, 4, 1), bitsliceget(i3, 6, 3));
    yt(out_idx+2) = bitconcat(bitsliceget(i3, 2, 1), i4);
    
    % Increment out_idx for next time through loop
    out_idx = out_idx + 3;
end

y = uint8(yt);

== matlab function eml_hdl_design_patterns/Misc/conditional_ops ==
  settings: fimath=|
      | fimath(...
      | 'RoundMode', 'floor',...
      | 'OverflowMode', 'wrap',...
      | 'ProductMode', 'FullPrecision', 'ProductWordLength', 32,...
      | 'SumMode', 'FullPrecision', 'SumWordLength', 32,...
      | 'CastBeforeSum', true)
  data: y output
function y = fcn
%%%%%%%%%%%%%%%%%%%%%%%%%%%%%%%%%%%%%%%%%%%%%%%%%%%%%%%%%%%%%%%
%%%%%%%%%%%%%%%% Recommendations for MATLAB/eML %%%%%%%%%%%%%%% 
%%%%%%%%%%%%%%%%%%%%%%%%%%%%%%%%%%%%%%%%%%%%%%%%%%%%%%%%%%%%%%%

% 
% Use the newer MATLAB operators || and &&, instead of the array versions 
% of these: | and &. The newer operators always short-circuit, not just 
% in if and while expressions. The newer operators force you to be clear 
% about your intention with respect to matrix expressions (including 
% empty ones) and you choose how to reduce the array expressions to 
% scalar ones that are unambiguous.
% 
% Logical variables have been part of MATLAB from the early days. 
% They are particularly useful in constructs involved flow-of-control, 
% such as if and while statements. But MATLAB, being an array-oriented 
% language, needs to deal with expressions following if and while that 
% might be of any size, including empty matrices. But sometimes users 
% get confused when two statements, seemingly the same, behave differently. 
% The understanding lies in the intersection of scalar expansion, 
% empty arrays, and logical operators, both short-circuit and elementwise.
% 
% Logical Operators, Scalar Expansion, and Empty Arrays
% 
% 
%
% 
% There are several concepts that might be helpful for understanding 
% this operator mystery.
% 
% 1) Empty arrays evaluate to false for the purposes of if and while.
%
% 2) The nonscalar | and & operators short-circuit in if and while expressions, 
%    but not otherwise in MATLAB.
%
% 3) It's best to feed if and while only scalar expressions. This means considering 
%    using the newer logical operators || and &&. 
%    These operators always short-circuit.
%
% 4) Use reduction operations explicitly to reduce expressions to scalar. 
%    Examples of these operations include 'all' and 'any'.
% 

% Use the || and && operators in expressions destined for if and while. 
% These expressions behave consistently, meaning they always short-circuit, 
% and are therefore easier to debug. They also force you to reduce 
% your expression to a scalar and it is easier to see what a 
% simple true or false means in the context of the flow-of-control. 

%%%%%%%%%%%%%%%%%%%%%%%%%%%%%%%%%%%%%%%%%%%%%%%%%%%%%%%%%%%
%%%%%%%%%%%%%%%% Recommendations for EML %%%%%%%%%%%%%%%%%% 
%%%%%%%%%%%%%%%%%%%%%%%%%%%%%%%%%%%%%%%%%%%%%%%%%%%%%%%%%%%

% eML forbids use of | and & in conditionals; try replacing
% || and && in the following conditional expressions with | and & and 
% see the eML lint messagages

% Non scalar expressions are not supported in conditionals in eML.
% if you remove 'all' from the following script you will get the error
%
% Expected a scalar. Non-scalar IF and WHILE are not supported.  
% Instead, use ALL to convert matrix logicals to their scalar equivalents.



y1 = false;
y2 = false;
y3 = false;
y4 = false;


if 4 || all([])
    y1 = true;
end

if all([]) || 4
    y2 = true;
end

dbg = 4 | any([]);

if dbg
    y3 = true;
end

dbg1 = 4 & any([]);

if dbg1
    y4 = true;
end

y = (y1 == true) && (y2 == true) && (y3 == true) && (y4 == false);

== matlab function eml_hdl_design_patterns/Word Twiddlers/rev32bits ==
  settings: fimath=|
      | fimath(...
      | 'RoundMode', 'floor',...
      | 'OverflowMode', 'wrap',...
      | 'ProductMode', 'FullPrecision', 'ProductWordLength', 32,...
      | 'SumMode', 'FullPrecision', 'SumWordLength', 32,...
      | 'CastBeforeSum', true)
  data: u input fixdt(0,32,0); y output
function y = fcn(u)

tn = u;

% const01 = hex2dec('55555555')
% const02 = hex2dec('33333333')
% const03 = hex2dec('0f0f0f0f')
% const04 = hex2dec('00ff00ff')
% const05 = hex2dec('0000ffff')
%
% const06 = hex2dec('aaaaaaaa')
% const07 = hex2dec('cccccccc')
% const08 = hex2dec('f0f0f0f0')
% const09 = hex2dec('ff00ff00')
% const10 = hex2dec('ffff0000')
%

const01 = fi(1431655765, numerictype(u), fimath(u));
const02 = fi(858993459, numerictype(u), fimath(u));
const03 = fi(252645135, numerictype(u), fimath(u));
const04 = fi(16711935, numerictype(u), fimath(u));
const05 = fi(65535, numerictype(u), fimath(u));

const06 = fi(2863311530, numerictype(u), fimath(u));
const07 = fi(3435973836, numerictype(u), fimath(u));
const08 = fi(4042322160, numerictype(u), fimath(u));
const09 = fi(4278255360, numerictype(u), fimath(u));
const10 = fi(4294901760, numerictype(u), fimath(u));


% fi_1 = fi(1, numerictype(u), fimath(u));
% fi_2 = fi(2, numerictype(u), fimath(u));
% fi_4 = fi(4, numerictype(u), fimath(u));
% fi_8 = fi(8, numerictype(u), fimath(u));
% fi_16 = fi(16, numerictype(u), fimath(u));
%
% fi_m1  = -fi_1;
% fi_m2  = -fi_2;
% fi_m4  = -fi_4;
% fi_m8  = -fi_8;
% fi_m16 = -fi_16;

% operation reverse stage1
tn = bitor(bitand(bitshift(tn, -1 )  , const01) , bitand(bitshift(tn, 1 ) , const06)) ;
% operation reverse stage2
tn = bitor(bitand(bitshift(tn, -2 )  , const02) , bitand(bitshift(tn, 2 ) , const07)) ;
% operation reverse stage3
tn = bitor(bitand(bitshift(tn, -4 )  , const03) , bitand(bitshift(tn, 4 ) , const08)) ;
% operation reverse stage4
tn = bitor(bitand(bitshift(tn, -8 )  , const04) , bitand(bitshift(tn, 8 ) , const09)) ;
% operation reverse stage5
tn = bitor(bitand(bitshift(tn, -16)  , const05) , bitand(bitshift(tn, 16) , const10)) ;

y = tn;

== matlab function eml_hdl_design_patterns/FSMs/detect even 1's and odd 0's ==
  settings: sampleTime=1
  settings: fimath=|
      | fimath(...
      | 'RoundMode', 'floor',...
      | 'OverflowMode', 'wrap',...
      | 'ProductMode', 'FullPrecision', 'ProductWordLength', 32,...
      | 'SumMode', 'FullPrecision', 'SumWordLength', 32,...
      | 'CastBeforeSum', true)
  data: u input uint8; y output; yc0 output; yc1 output
function [y,yc0,yc1] = fcn(u) 
%% This function sets the output 'y' if 
%% even number of 1's and odd number of 0's are detected.


persistent state;
persistent cnt0; % Counting 0's
persistent cnt1; % Counting 1's

if(isempty(state))
    state = fi(0,0,2,0);  % ufix2(0)
    cnt0 = uint8(0);
    cnt1 = uint8(0);
end

y = uint8(0);

switch(uint8(state))
    case uint8(0)
        if(u == 0)
            state = fi(3,0,2,0);
            cnt0 = cnt0 + 1;
            y = uint8(1);   %% even 1's and odd 0's detected
        else
            state = fi(1,0,2,0);
            cnt1 = cnt1 + 1;
        end
    case uint8(1)
        if(u == 0)
            state = fi(2,0,2,0);
            cnt0 = cnt0 + 1;
        else
            state = fi(0,0,2,0);
            cnt1 = cnt1 + 1;
        end
    case uint8(2)
        if(u == 0)
            state = fi(1,0,2,0);
            cnt0 = cnt0 + 1;
        else
            state = fi(3,0,2,0);
            cnt1 = cnt1 + 1;
            y = uint8(1);   %% even 1's and odd 0's detected
        end
    case uint8(3)
        if(u == 0)
            state = fi(0,0,2,0);
            cnt0 = cnt0 + 1;
        else
            state = fi(2,0,2,0);
            cnt1 = cnt1 + 1;
        end
end

yc0 = cnt0;
yc1 = cnt1;

== matlab function eml_hdl_design_patterns/Sequences/stepseq ==
  settings: fimath=|
      | fimath(...
      | 'RoundMode', 'floor',...
      | 'OverflowMode', 'wrap',...
      | 'ProductMode', 'FullPrecision', 'ProductWordLength', 32,...
      | 'SumMode', 'FullPrecision', 'SumWordLength', 32,...
      | 'CastBeforeSum', true)
  data: x output; n output
function [x,n] = fcn
% Generates x(n) = u(n-n0); n1 <= n,n0 <= n2
% [x,n] = stepseq(n0,n1,n2)
%

n1 = 0;
n2 = 99;
n0 = 50;

if ((n0 < n1) || (n0 > n2) || (n1 > n2))
	error('arguments must satisfy n1 <= n0 <= n2')
end

n = fi(n1:n2, 0, 10, 2);

%x = [zeros(1,(n0-n1)), ones(1,(n2-n0+1))];
x = (n-n0) > 0;
